simulink model "avc_simulation"  (R2025b)
settings: Solver=VariableStepAuto  StartTime=0.0  StopTime=10.0  RelTol=1e-3
values from neighbouring files (symbols this model uses):
  Ad = sys_discrete.A    [program.m]
  Bd = sys_discrete.B    [program.m]
  Cd = sys_discrete.C    [program.m]
  Dd = sys_discrete.D    [program.m]
  f_bpf = 80    [program.m]
  Ts = 1/2000    (= 0.0005)    [ekf_algorithm.m]    (also in program.m)
undefined symbols (not defined in the file or in its folder): den_s, dspblkCoreblockFVToolHelper, gcbh, num_s
libraries: simulink x1, dspadpt3 x1
settings Model: Creator=angeloskamariadis  LastModifiedBy=angeloskamariadis

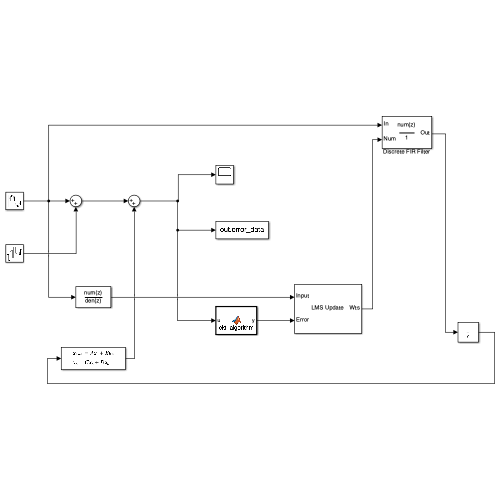
[thumbnail: Simulink's stored preview of the top-level diagram]
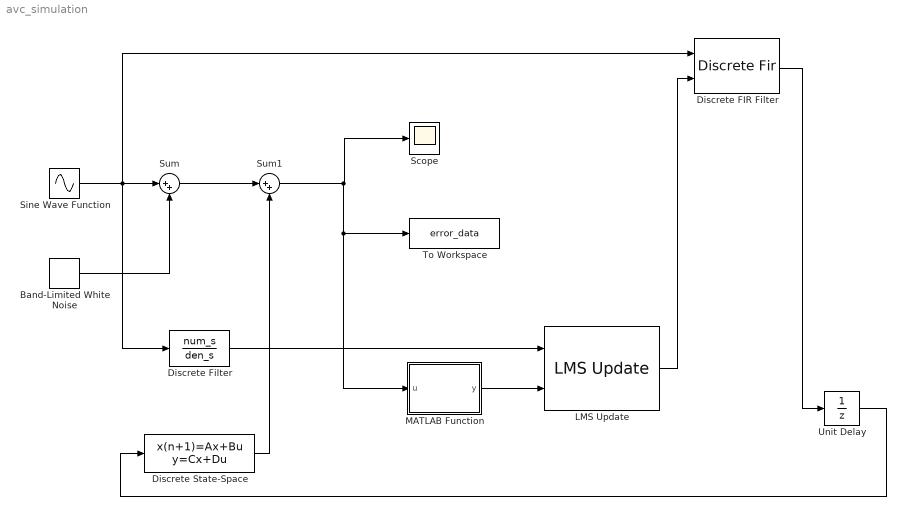
== system avc_simulation ==
  Band-Limited White Noise : simulink/Sources/Band-Limited White Noise  Cov=1e-5  Ts=Ts  seed=[23341]
  Discrete FIR Filter : DiscreteFir  LoadFcn=dspblkCoreblockFVToolHelper(gcbh,'load');  CoefSource=Input port  InputProcessing=Columns as channels (frame based)
      settings: CopyFcn=dspblkCoreblockFVToolHelper(gcbh,'copy');  DeleteFcn=dspblkCoreblockFVToolHelper(gcbh,'close');  ModelCloseFcn=dspblkCoreblockFVToolHelper(gcbh,'close');  PreSaveFcn=dspblkCoreblockFVToolHelper(gcbh,'presave');  PostSaveFcn=dspblkCoreblockFVToolHelper(gcbh,'postsave');  CloseFcn=dspblkCoreblockFVToolHelper(gcbh,'close');  InputPortMap=u0,u1
  Discrete Filter : DiscreteFilter  LoadFcn=dspblkCoreblockFVToolHelper(gcbh,'load');  Numerator=num_s  Denominator=den_s
      settings: CopyFcn=dspblkCoreblockFVToolHelper(gcbh,'copy');  DeleteFcn=dspblkCoreblockFVToolHelper(gcbh,'close');  ModelCloseFcn=dspblkCoreblockFVToolHelper(gcbh,'close');  PreSaveFcn=dspblkCoreblockFVToolHelper(gcbh,'presave');  PostSaveFcn=dspblkCoreblockFVToolHelper(gcbh,'postsave');  CloseFcn=dspblkCoreblockFVToolHelper(gcbh,'close');
  Discrete State-Space : DiscreteStateSpace  A=Ad  B=Bd  C=Cd  D=Dd  SampleTime=Ts
  LMS Update : dspadpt3/LMS Update  Method=Normalized LMS  Length=64  NumFilters=1  StepSizeSource=Property  StepSize=0.1  LeakageFactor=1.0  InitialConditions=0  AdaptiveFilterMode=Tapped delay-line FIR filter  EnableAdaptInput=off  EnableResetInput=off  SimulateUsing=Interpreted execution
  MATLAB Function : MATLAB Function  TreatAsAtomicUnit=on
  Scope : Scope
      settings: ActiveDisplayYMinimum=-291.36805730862613  ActiveDisplayYMaximum=313.49855912087446
  Sine Wave Function : Sin  Amplitude=10  Frequency=2*pi*f_bpf  SampleTime=Ts
  Sum : Sum  Inputs=|++
  Sum1 : Sum  Inputs=|++
  To Workspace : ToWorkspace  VariableName=error_data  SampleTime=-1
  Unit Delay : UnitDelay  SampleTime=-1  HasFrameUpgradeWarning=on
  wires:
  Sine Wave Function/1 -> Discrete FIR Filter/1, Discrete Filter/1, Sum/1
  Band-Limited White Noise/1 -> Sum/2
  Sum/1 -> Sum1/1
  Discrete State-Space/1 -> Sum1/2
  Sum1/1 -> To Workspace/1, MATLAB Function/1(u), Scope/1
  Unit Delay/1 -> Discrete State-Space/1
  Discrete Filter/1 -> LMS Update/1
  MATLAB Function/1(y) -> LMS Update/2
  Discrete FIR Filter/1 -> Unit Delay/1
  LMS Update/1 -> Discrete FIR Filter/2

== matlab function avc_simulation/MATLAB Function ==
  data: u input; y output
function y = ekf_algorithm(u)

persistent x_hat P Q R F_k H_k

if isempty(x_hat)
    x_hat = [0; 0]; 
    P = [1, 0; 
         0, 1];
    Q = [1e-6, 0; 
         0,    1e-6]; 
    R = 1e-2; 
    m = 0.5; k = 5000; c = 2.5; Ts = 1/2000;
    Ac = [0,       1; 
         -k/m, -c/m];
    F_k = expm(Ac * Ts); 
    
    H_k = [1, 0];
end

% -------------------------------------------------------------------------
% EKF PREDICT STEP (Priori)
% -------------------------------------------------------------------------
x_hat_minus = F_k * x_hat; 
P_minus = (F_k * P * F_k') + Q;

% -------------------------------------------------------------------------
% EKF UPDATE STEP (Posteriori)
% -------------------------------------------------------------------------
S = (H_k * P_minus * H_k') + R;
K = P_minus * H_k' / S;
x_hat = x_hat_minus + K * (u - (H_k * x_hat_minus));
I_KH = eye(2) - (K * H_k);
P = (I_KH * P_minus * I_KH') + (K * R * K');

% -------------------------------------------------------------------------
% OUTPUT TO DSP
% -------------------------------------------------------------------------
y = H_k * x_hat;

end
